simulink model "bms_twin_ekf"  (R2025b)
settings: Solver=FixedStepDiscrete  StartTime=0.0  StopTime=t_stop  FixedStep=Ts  RelTol=1e-3
values from neighbouring files (symbols this model uses):
  Age_Q = 1    [bms_init.m]    (also in test_ml_soh.m = soh)
  Age_R = 1    [bms_init.m]    (also in test_ml_soh.m = rr)
  bias_i = P.bias_i    [bms_init.m]
  Bms_Q = 1    [bms_init.m]    (also in test_ml_soh.m = cfg{b,2})
  Bms_R = 1    [bms_init.m]    (also in test_ml_soh.m = cfg{b,3})
  Can_dur = Inf    (= inf)    [bms_init.m]    (also in test_can_monitor.m = S{s,6})
  Can_mode = 0    [bms_init.m]    (also in test_can_monitor.m = S{s,3})
  Can_msg = 3    [bms_init.m]    (also in test_can_monitor.m = S{s,4})
  Can_t = 600    [bms_init.m]    (also in test_can_monitor.m = S{s,5})
  Dec_on = 0    [bms_init.m]    (also in test_can_monitor.m = 1; test_decision.m = dec)
  Diag_on = 1    [bms_init.m]    (also in test_sensor_faults.m = dg)
  Fault_mode = 0    [bms_init.m]    (also in test_decision.m = S{s,7}; test_sensor_faults.m = cases{c,1})
  Fault_t = 1200    [bms_init.m]
  I_allow_chg = P.i_max_chg * P.Np    [bms_init.m]    (also in build_bms_model.m = I_fix_chg; decision_logic.m = D.i_chg)
  I_allow_dis = P.i_max_dis * P.Np    [bms_init.m]    (also in build_bms_model.m = I_fix_dis; decision_logic.m = D.i_dis)
  Rint_den0 = 0    [bms_init.m]    (also in test_ml_soh.m)
  Rint_num0 = 0    [bms_init.m]    (also in test_ml_soh.m)
  Ru_factor = 1    [bms_init.m]    (also in scenarios.m = sc(k).Ru; test_decision.m = S{s,4}; test_sensor_faults.m = SC{s,3}; test_thermal_observer.m = SC{s,3})
  seed_i = 22    [bms_init.m]    (also in test_ml_soh.m = 201)
  seed_t = 33    [bms_init.m]    (also in test_ml_soh.m = 202)
  seed_v = 11    [bms_init.m]    (also in test_ml_soh.m = 200)
  seed_vmax = 55    [bms_init.m]
  seed_vmin = 44    [bms_init.m]
  sig_i = P.sig_i    [bms_init.m]
  sig_t = P.sig_t    [bms_init.m]
  sig_v = P.sig_v    [bms_init.m]
  sig_vc = 0.005    [bms_init.m]
  SOC0 = P.soc0    [bms_init.m]    (also in scenarios.m = sc(k).SOC0; test_decision.m = S{s,5}; test_sensor_faults.m = SC{s,4}; test_week1_extras.m = 0.4)
  T_amb = 25    [bms_init.m]    (also in scenarios.m = sc(k).T_amb; test_decision.m = S{s,3}; test_sensor_faults.m = SC{s,2}; test_thermal_observer.m = SC{s,2})
  Ts = P.Ts    [bms_init.m]
  Usage = [0 0 25 0.5 1]    [bms_init.m]    (also in test_ml_soh.m = C{c,4})
  Weak_on = 0    [bms_init.m]    (also in test_decision.m = S{s,6}; test_week1_extras.m = k - 1)
settings Model: Creator=berka  LastModifiedBy=berka

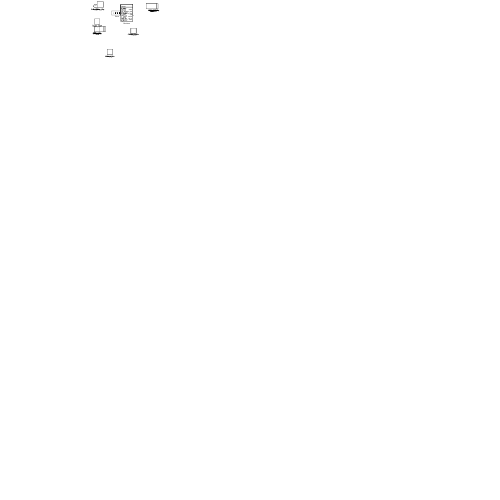
[thumbnail: Simulink's stored preview of the top-level diagram]
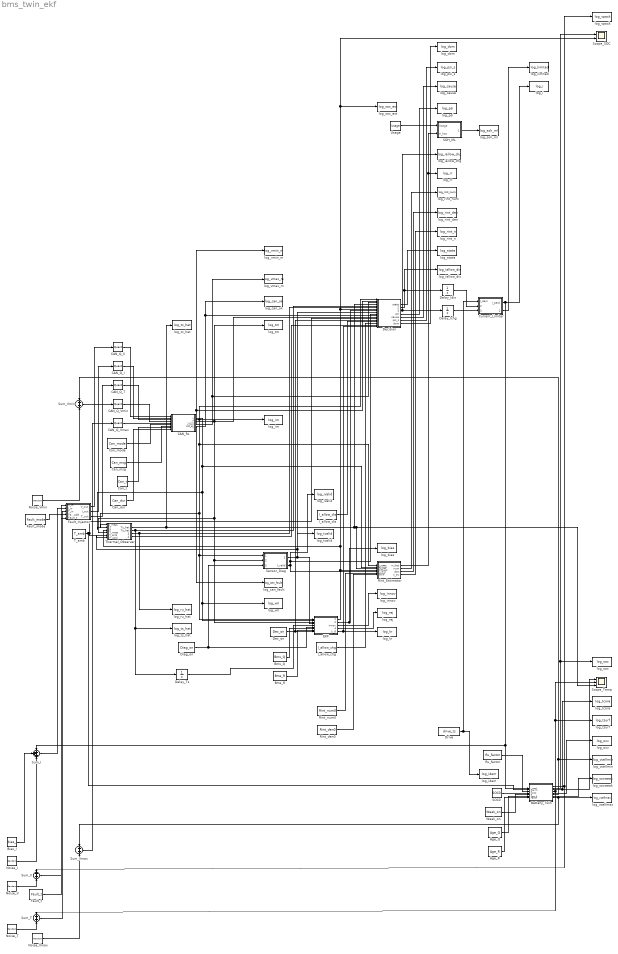
== system bms_twin_ekf ==
  Age_Q : Constant  Value=Age_Q
  Age_R : Constant  Value=Age_R
  Battery_Twin : MATLAB Function  TreatAsAtomicUnit=on
  Bias_I : Constant  Value=bias_i
  Bms_Q : Constant  Value=Bms_Q
  Bms_R : Constant  Value=Bms_R
  CAN_Q_I : Quantizer  QuantizationInterval=lsb_i
  CAN_Q_T : Quantizer  QuantizationInterval=lsb_t
  CAN_Q_V : Quantizer  QuantizationInterval=lsb_v
  CAN_Q_Vmax : Quantizer  QuantizationInterval=lsb_vc
  CAN_Q_Vmin : Quantizer  QuantizationInterval=lsb_vc
  CAN_Rx : MATLAB Function  TreatAsAtomicUnit=on
  Can_dur : Constant  Value=Can_dur
  Can_mode : Constant  Value=Can_mode
  Can_msg : Constant  Value=Can_msg
  Can_t : Constant  Value=Can_t
  Current_Limiter : MATLAB Function  TreatAsAtomicUnit=on
  Dec_on : Constant  Value=Dec_on
  Decision : MATLAB Function  TreatAsAtomicUnit=on
  Delay_Ichg : UnitDelay  InitialCondition=I_allow_chg*(1-Dec_on)  SampleTime=Ts  HasFrameUpgradeWarning=on
  Delay_Idis : UnitDelay  InitialCondition=I_allow_dis*(1-Dec_on)  SampleTime=Ts  HasFrameUpgradeWarning=on
  Delay_Ts : UnitDelay  InitialCondition=T_amb  SampleTime=Ts  HasFrameUpgradeWarning=on
  Diag_on : Constant  Value=Diag_on
  Drive : FromWorkspace  VariableName=drive_ts  SampleTime=Ts  Interpolate=off  OutputAfterFinalValue=Holding final value
  EKF : MATLAB Function  TreatAsAtomicUnit=on
  Fault_Injector : MATLAB Function  TreatAsAtomicUnit=on
  Fault_mode : Constant  Value=Fault_mode
  Fault_t : Constant  Value=Fault_t
  I_allow_chg : Constant  Value=I_allow_chg
  I_allow_dis : Constant  Value=I_allow_dis
  Noise_I : RandomNumber  Variance=sig_i^2  Seed=seed_i  SampleTime=Ts
  Noise_T : RandomNumber  Variance=sig_t^2  Seed=seed_t  SampleTime=Ts
  Noise_V : RandomNumber  Variance=sig_v^2  Seed=seed_v  SampleTime=Ts
  Noise_Vmax : RandomNumber  Variance=sig_vc^2  Seed=seed_vmax  SampleTime=Ts
  Noise_Vmin : RandomNumber  Variance=sig_vc^2  Seed=seed_vmin  SampleTime=Ts
  Rint_Estimator : MATLAB Function  TreatAsAtomicUnit=on
  Rint_den0 : Constant  Value=Rint_den0
  Rint_num0 : Constant  Value=Rint_num0
  Ru_factor : Constant  Value=Ru_factor
  SOC0 : Constant  Value=SOC0
  SOH_ML : MATLAB Function  TreatAsAtomicUnit=on
  Scope_SOC : Scope  NumInputPorts=2
  Scope_Temp : Scope  NumInputPorts=3
  Sensor_Diag : MATLAB Function  TreatAsAtomicUnit=on
  Sum_I : Sum  Inputs=+++
  Sum_T : Sum
  Sum_V : Sum
  Sum_Vmax : Sum
  Sum_Vmin : Sum
  T_amb : Constant  Value=T_amb
  Thermal_Observer : MATLAB Function  TreatAsAtomicUnit=on
  Usage : Constant  Value=Usage
  Weak_on : Constant  Value=Weak_on
  log_bias : ToWorkspace  VariableName=log_bias  SampleTime=-1
  log_can_fault : ToWorkspace  VariableName=log_can_fault  SampleTime=-1
  log_can_ok : ToWorkspace  VariableName=log_can_ok  SampleTime=-1
  log_cause : ToWorkspace  VariableName=log_cause  SampleTime=-1
  log_dom : ToWorkspace  VariableName=log_dom  SampleTime=-1
  log_i : ToWorkspace  VariableName=log_i  SampleTime=-1
  log_iallow_chg : ToWorkspace  VariableName=log_iallow_chg  SampleTime=-1
  log_iallow_dis : ToWorkspace  VariableName=log_iallow_dis  SampleTime=-1
  log_idem : ToWorkspace  VariableName=log_idem  SampleTime=-1
  log_im : ToWorkspace  VariableName=log_im  SampleTime=-1
  log_innov : ToWorkspace  VariableName=log_innov  SampleTime=-1
  log_ivalid : ToWorkspace  VariableName=log_ivalid  SampleTime=-1
  log_kr : ToWorkspace  VariableName=log_kr  SampleTime=-1
  log_limited : ToWorkspace  VariableName=log_limited  SampleTime=-1
  log_ocv : ToWorkspace  VariableName=log_ocv  SampleTime=-1
  log_psi : ToWorkspace  VariableName=log_psi  SampleTime=-1
  log_psi_s : ToWorkspace  VariableName=log_psi_s  SampleTime=-1
  log_rej : ToWorkspace  VariableName=log_rej  SampleTime=-1
  log_rint_den : ToWorkspace  VariableName=log_rint_den  SampleTime=-1
  log_rint_n : ToWorkspace  VariableName=log_rint_n  SampleTime=-1
  log_rint_num : ToWorkspace  VariableName=log_rint_num  SampleTime=-1
  log_rr : ToWorkspace  VariableName=log_rr  SampleTime=-1
  log_ru_hat : ToWorkspace  VariableName=log_ru_hat  SampleTime=-1
  log_soc : ToWorkspace  VariableName=log_soc  SampleTime=-1
  log_soc_est : ToWorkspace  VariableName=log_soc_est  SampleTime=-1
  log_socweak : ToWorkspace  VariableName=log_socweak  SampleTime=-1
  log_soh_ml : ToWorkspace  VariableName=log_soh_ml  SampleTime=-1
  log_state : ToWorkspace  VariableName=log_state  SampleTime=-1
  log_tc_hat : ToWorkspace  VariableName=log_tc_hat  SampleTime=-1
  log_tcore : ToWorkspace  VariableName=log_tcore  SampleTime=-1
  log_tm : ToWorkspace  VariableName=log_tm  SampleTime=-1
  log_ts_hat : ToWorkspace  VariableName=log_ts_hat  SampleTime=-1
  log_tsurf : ToWorkspace  VariableName=log_tsurf  SampleTime=-1
  log_tvalid : ToWorkspace  VariableName=log_tvalid  SampleTime=-1
  log_vcellmax : ToWorkspace  VariableName=log_vcellmax  SampleTime=-1
  log_vcellmin : ToWorkspace  VariableName=log_vcellmin  SampleTime=-1
  log_vm : ToWorkspace  VariableName=log_vm  SampleTime=-1
  log_vmax_m : ToWorkspace  VariableName=log_vmax_m  SampleTime=-1
  log_vmin_m : ToWorkspace  VariableName=log_vmin_m  SampleTime=-1
  log_vpack : ToWorkspace  VariableName=log_vpack  SampleTime=-1
  wires:
  Decision/3(I_allow_chg) -> Delay_Ichg/1, log_iallow_chg/1
  EKF/1(SOC_est) -> log_soc_est/1, Scope_SOC/2, Decision/7(SOC_est), Thermal_Observer/3(SOC_est), Rint_Estimator/4(SOC_est)
  Sum_Vmax/1 -> CAN_Q_Vmax/1
  Noise_Vmin/1 -> Sum_Vmin/2
  Decision/7(dom) -> log_dom/1
  Bias_I/1 -> Sum_I/2
  Noise_T/1 -> Sum_T/2
  Delay_Ts/1 -> EKF/5(Ts_hat_prev)
  Noise_V/1 -> Sum_V/2
  Noise_I/1 -> Sum_I/3
  Fault_mode/1 -> Fault_Injector/4(Fault_mode)
  Decision/2(I_allow_dis) -> log_iallow_dis/1, Delay_Idis/1
  Bms_R/1 -> EKF/8(R_scale)
  Diag_on/1 -> Sensor_Diag/3(Diag_on), EKF/6(Gate_on)
  Sum_V/1 -> Fault_Injector/1(V_in)
  CAN_Q_Vmax/1 -> CAN_Rx/5(Vmax_in)
  EKF/4(rejected) -> log_rej/1
  Current_Limiter/1(I_pack) -> Sum_I/1, Battery_Twin/1(I_pack), log_i/1
  Sum_I/1 -> Fault_Injector/2(I_in)
  Bms_Q/1 -> EKF/7(Q_scale)
  Rint_Estimator/1(rr_hat) -> SOH_ML/2(rr_hat), log_rr/1
  I_allow_chg/1 -> Decision/16(I_fix_chg)
  Fault_t/1 -> Fault_Injector/5(Fault_t)
  EKF/3(innov) -> log_innov/1
  Fault_Injector/1(V_out) -> CAN_Q_V/1
  Sum_T/1 -> Fault_Injector/3(T_in)
  Noise_Vmax/1 -> Sum_Vmax/2
  CAN_Q_Vmin/1 -> CAN_Rx/4(Vmin_in)
  Sum_Vmin/1 -> CAN_Q_Vmin/1
  Fault_Injector/2(I_out) -> CAN_Q_I/1
  Fault_Injector/3(T_out) -> CAN_Q_T/1
  I_allow_dis/1 -> Decision/15(I_fix_dis)
  Thermal_Observer/2(Ts_hat) -> log_ts_hat/1, Delay_Ts/1, Decision/5(Ts_hat)
  T_amb/1 -> Decision/13(T_amb), Thermal_Observer/5(T_amb), Battery_Twin/2(T_amb)
  CAN_Q_V/1 -> CAN_Rx/1(V_in)
  Weak_on/1 -> Battery_Twin/5(Weak_on)
  CAN_Q_I/1 -> CAN_Rx/2(I_in)
  CAN_Rx/1(V) -> EKF/2(V_meas), log_vm/1, Thermal_Observer/2(V_meas), Rint_Estimator/2(V_meas)
  CAN_Q_T/1 -> CAN_Rx/3(T_in)
  Usage/1 -> SOH_ML/1(Usage)
  Rint_num0/1 -> Rint_Estimator/6(num0)
  Can_t/1 -> CAN_Rx/8(Can_t)
  Can_mode/1 -> CAN_Rx/6(Can_mode)
  Rint_den0/1 -> Rint_Estimator/7(den0)
  CAN_Rx/4(V_min) -> Decision/2(V_min), log_vmin_m/1
  Dec_on/1 -> Decision/14(Dec_on), EKF/9(Zero_on)
  Can_dur/1 -> CAN_Rx/9(Can_dur)
  Can_msg/1 -> CAN_Rx/7(Can_msg)
  Thermal_Observer/1(Tc_hat) -> Scope_Temp/3, Rint_Estimator/3(Tc_hat), Decision/4(Tc_hat), log_tc_hat/1
  Thermal_Observer/3(Ru_hat) -> Decision/6(Ru_hat), log_ru_hat/1
  Thermal_Observer/4(T_anom) -> Decision/17(T_anom)
  Rint_Estimator/3(den) -> log_rint_den/1
  CAN_Rx/2(I) -> EKF/1(I_meas), Sensor_Diag/1(I_meas), Thermal_Observer/1(I_meas), Rint_Estimator/1(I_meas), Decision/1(I_meas), log_im/1
  CAN_Rx/3(T) -> EKF/3(T_meas), Sensor_Diag/2(T_meas), Thermal_Observer/4(T_meas), Decision/12(T_meas), log_tm/1
  CAN_Rx/5(V_max) -> Decision/3(V_max), log_vmax_m/1
  CAN_Rx/6(CAN_ok) -> Decision/11(CAN_ok), log_can_ok/1
  CAN_Rx/7(can_fault) -> log_can_fault/1
  Sensor_Diag/1(T_valid) -> Decision/9(T_valid), EKF/4(T_valid), log_tvalid/1, Thermal_Observer/6(T_valid)
  Sensor_Diag/2(I_valid) -> Decision/10(I_valid), log_ivalid/1, Rint_Estimator/5(I_valid)
  EKF/2(bias_est) -> Decision/8(bias_est), log_bias/1
  EKF/5(k_R) -> Decision/18(k_R), log_kr/1
  Decision/1(state) -> log_state/1
  Decision/4(psi) -> log_psi/1
  Decision/5(cause) -> log_cause/1
  Decision/6(psi_s) -> log_psi_s/1
  Rint_Estimator/2(num) -> log_rint_num/1
  Rint_Estimator/4(n_ev) -> log_rint_n/1
  SOH_ML/1(SOH_hat) -> log_soh_ml/1
  Delay_Idis/1 -> Current_Limiter/2(I_allow_dis)
  Delay_Ichg/1 -> Current_Limiter/3(I_allow_chg)
  Drive/1 -> Current_Limiter/1(I_dem), log_idem/1
  Current_Limiter/2(limited) -> log_limited/1
  Ru_factor/1 -> Battery_Twin/3(Ru_factor)
  SOC0/1 -> Battery_Twin/4(SOC0)
  Age_Q/1 -> Battery_Twin/6(Age_Q)
  Age_R/1 -> Battery_Twin/7(Age_R)
  Battery_Twin/1(V_pack) -> Sum_V/1, log_vpack/1
  Battery_Twin/2(SOC) -> log_soc/1, Scope_SOC/1
  Battery_Twin/3(T_core) -> log_tcore/1, Scope_Temp/1
  Battery_Twin/4(T_surf) -> log_tsurf/1, Scope_Temp/2, Sum_T/1
  Battery_Twin/5(OCV_pack) -> log_ocv/1
  Battery_Twin/6(V_cell_min) -> Sum_Vmin/1, log_vcellmin/1
  Battery_Twin/7(SOC_weak) -> log_socweak/1
  Battery_Twin/8(V_cell_max) -> Sum_Vmax/1, log_vcellmax/1

== matlab function bms_twin_ekf/EKF ==
  data: I_meas input; SOC_est output; V_meas input; T_meas input; T_valid input; Ts_hat_prev input; Gate_on input; Q_scale input; R_scale input; Zero_on input; bias_est output; innov output; rejected output; k_R output
function [SOC_est, bias_est, innov, rejected, k_R] = ekf_blk(I_meas, V_meas, T_meas, T_valid, Ts_hat_prev, Gate_on, Q_scale, R_scale, Zero_on)
%#codegen
[SOC_est, bias_est, innov, rejected, k_R] = ekf_soc(I_meas, V_meas, T_meas, T_valid, Ts_hat_prev, Gate_on, Q_scale, R_scale, Zero_on);
end

== matlab function bms_twin_ekf/Thermal_Observer ==
  data: I_meas input; Tc_hat output; V_meas input; SOC_est input; T_meas input; T_amb input; T_valid input; Ts_hat output; Ru_hat output; T_anom output
function [Tc_hat, Ts_hat, Ru_hat, T_anom] = thobs_blk(I_meas, V_meas, SOC_est, T_meas, T_amb, T_valid)
%#codegen
[Tc_hat, Ts_hat, Ru_hat, T_anom] = thermal_observer(I_meas, V_meas, SOC_est, T_meas, T_amb, T_valid);
end

== matlab function bms_twin_ekf/Rint_Estimator ==
  data: I_meas input; rr_hat output; V_meas input; Tc_hat input; SOC_est input; I_valid input; num0 input; den0 input; num output; den output; n_ev output
function [rr_hat, num, den, n_ev] = rint_blk(I_meas, V_meas, Tc_hat, SOC_est, I_valid, num0, den0)
%#codegen
[rr_hat, num, den, n_ev] = rint_estimator(I_meas, V_meas, Tc_hat, SOC_est, I_valid, num0, den0);
end

== matlab function bms_twin_ekf/SOH_ML ==
  data: Usage input; SOH_hat output; rr_hat input
function SOH_hat = soh_blk(Usage, rr_hat)
%#codegen
% Usage = [efc days T_mean SOC_mean DoD]: BMS lifetime counters (EEPROM in HIL)
SOH_hat = soh_tree(Usage(1), Usage(2), Usage(3), Usage(4), Usage(5), rr_hat);
end

== matlab function bms_twin_ekf/Decision ==
  data: I_meas input; state output; V_min input; V_max input; Tc_hat input; Ts_hat input; Ru_hat input; SOC_est input; bias_est input; T_valid input; I_valid input; CAN_ok input; T_meas input; T_amb input; Dec_on input; I_fix_dis input; I_fix_chg input; T_anom input; k_R input; I_allow_dis output; I_allow_chg output; psi output; cause output; psi_s output; dom output
function [state, I_allow_dis, I_allow_chg, psi, cause, psi_s, dom] = dec_blk(I_meas, V_min, V_max, Tc_hat, Ts_hat, Ru_hat, SOC_est, bias_est, T_valid, I_valid, CAN_ok, T_meas, T_amb, Dec_on, I_fix_dis, I_fix_chg, T_anom, k_R)
%#codegen
if Dec_on > 0.5
    [state, I_allow_dis, I_allow_chg, psi, cause, psi_s, dom] = decision_logic(I_meas, V_min, V_max, Tc_hat, Ts_hat, Ru_hat, SOC_est, bias_est, T_valid, I_valid, CAN_ok, T_meas, T_amb, T_anom, k_R);
else
    state = 1; I_allow_dis = I_fix_dis; I_allow_chg = I_fix_chg; psi = 0; cause = 0; psi_s = 0; dom = 0;
end
end

== matlab function bms_twin_ekf/Battery_Twin ==
  data: I_pack input; V_pack output; T_amb input; Ru_factor input; SOC0 input; Weak_on input; Age_Q input; Age_R input; SOC output; T_core output; T_surf output; OCV_pack output; V_cell_min output; SOC_weak output; V_cell_max output
function [V_pack, SOC, T_core, T_surf, OCV_pack, V_cell_min, SOC_weak, V_cell_max] = twin_blk(I_pack, T_amb, Ru_factor, SOC0, Weak_on, Age_Q, Age_R)
%#codegen
[V_pack, SOC, T_core, T_surf, OCV_pack, V_cell_min, SOC_weak, V_cell_max] = battery_twin(I_pack, T_amb, Ru_factor, SOC0, Weak_on, Age_Q, Age_R);
end

== matlab function bms_twin_ekf/Current_Limiter ==
  data: I_dem input; I_pack output; I_allow_dis input; I_allow_chg input; limited output
function [I_pack, limited] = lim_blk(I_dem, I_allow_dis, I_allow_chg)
%#codegen
[I_pack, limited] = current_limiter(I_dem, I_allow_dis, I_allow_chg);
end

== matlab function bms_twin_ekf/Fault_Injector ==
  data: V_in input; V_out output; I_in input; T_in input; Fault_mode input; Fault_t input; I_out output; T_out output
function [V_out, I_out, T_out] = fault_blk(V_in, I_in, T_in, Fault_mode, Fault_t)
%#codegen
[V_out, I_out, T_out] = fault_injector(V_in, I_in, T_in, Fault_mode, Fault_t);
end

== matlab function bms_twin_ekf/CAN_Rx ==
  data: V_in input; V output; I_in input; T_in input; Vmin_in input; Vmax_in input; Can_mode input; Can_msg input; Can_t input; Can_dur input; I output; T output; V_min output; V_max output; CAN_ok output; can_fault output
function [V, I, T, V_min, V_max, CAN_ok, can_fault] = canrx_blk(V_in, I_in, T_in, Vmin_in, Vmax_in, Can_mode, Can_msg, Can_t, Can_dur)
%#codegen
[V, I, T, V_min, V_max, CAN_ok, can_fault] = can_rx(V_in, I_in, T_in, Vmin_in, Vmax_in, Can_mode, Can_msg, Can_t, Can_dur);
end

== matlab function bms_twin_ekf/Sensor_Diag ==
  data: I_meas input; T_valid output; T_meas input; Diag_on input; I_valid output
function [T_valid, I_valid] = diag_blk(I_meas, T_meas, Diag_on)
%#codegen
[T_valid, I_valid] = sensor_diag(I_meas, T_meas, Diag_on);
end
